simulink model "test_SimulinkMdl2_qLPVMPCbeta_UIO_testOL2"  (R2019b)
settings: Solver=FixedStepAuto  StartTime=0.0  StopTime=400  FixedStep=DT  RelTol=1e-3
values from neighbouring files (symbols this model uses):
  beta = [-0.13962634015954636; -0.1361356816555577; -0.13264502315156904;          -0.12915436464758037; -0.12566370614359171; -0.12217304763960307;          -0.11868238913561441; -0.11519173063162574; -0.11170107212763709;          -0.10821041362364842; -0.10471975511965977; -0.10122909661567112;          -0.097738438111682452; -0.094247779607693788; -0.09075712110370511;          -0.087266462599716474;  ...(+3598 chars)    [MdlMFile.m]
  betaLUT = 0.0 0.064193209888351435 0.11259119004615419 0.14929546421559495 0.18081611050661253 0.20926497731412011 0.23701571242082992 0.26197392072434883 0.28536133270107289 0.30770154712660031 0.32934362985133 0.35028758087526196 0.37035886727319672 0.38973202197033374 0.40858157789187255    [DD_test.sldd]    (also in exUIO_WECS.m = unique(Lin_points.Pitch))
  Cq = saveVarsMat.Cq    [MdlMFile.m]
  Ct = saveVarsMat.Ct    [MdlMFile.m]
  DT = 0.008    [LUTMFile.m]    (also in UIOLinestTr.m; exUIO_WECS.m; getFictInputMatricesOrd3M.m; initWorkspace.m)
  in1 = [Tr,Tg]    [UIOLinestTr.m]    (also in exUIO_WECS.m = [d,u1,u2])
  lambda = [0; 0.1; 0.2; 0.30000000000000004; 0.4; 0.5; 0.60000000000000009;            0.70000000000000007; 0.8; 0.9; 1; 1.1; 1.2000000000000002; 1.3;            1.4000000000000001; 1.5; 1.6; 1.7000000000000002; 1.8; 1.9000000000000001;            2; 2.1; 2.2; 2.3000000000000003; 2.4000000000000004; 2.5; 2.6;            2.7; 2.8000000000000003; 2.9000000000000004; 3; 3.1; 3.2; 3.3000000000000003;            ...(+1285 chars)    [MdlMFile.m]    (also in exLQR_hamiltonian.m = -10; koopmanKhalil.m = 1)
  lambdaCqVecLUT = 0.0 6.127061506348616E-5 0.00012254123012697232 0.00018381184519045848 0.00024508246025394464 0.00030635307531743077 0.00036762369038091696 0.00042889430544440315 0.00049016492050788928 0.00055143553557137541 0.00061270615063486154 0.00067397676569834778 0.00073524738076183392 0.00079651799582532 0.00085778861088880629 0.00091905922595229242 0.00098032984101577856 0.0010416004560792648 0.001102871    [DD_test.sldd]    (also in exUIO_WECS.m = lambdaCqVecMin : dLlambdaCqVec:lambdaCqVecMax)
  lambdaTildaMat = 14.419529569316524 14.349603210880673 12.133085869773012 9.9 8.4 7.3000000000000007 6.5 5.8000000000000007 5.4 4.9 4.6000000000000005 4.3 4.1000000000000005 3.9000000000000004 3.7 13.719392614649337 13.574357234178933 11.313379017594022 9.2598290519250313 7.9268106449449158 6.9824653636911407 6.2259000594299776 5.6530125740384722 5.1921371802911152 4.81807621242771 4.4910785109643978 4.22716815598    [DD_test.sldd]    (also in exUIO_WECS.m = lambdaCqVecMax *ones(size(lambdaCqMat)))
  Lin_points = 0.74811652133345019 0.78122947334555715 0.82586806925039735 0.88042797952230989 0.94564154658981237 1.06231329175348 1.1780905557148451 1.2402773842094346 1.254474305465946 1.2544764615597244 1.2544775037226534 1.2544778841663968 1.2544780221694662 1.2544779823335293 1.254477987181289 1.2544781738200332 1.254478189259095 1.2544780953600987 1.2544781548505395 1.2544783366942183 1.2544785605869417 1    [DD_test.sldd]    (also in LinPointsMFile.m = struct)
  multTau = 0.02    [UIOLinestTr.m]    (also in exUIO_WECS.m = 1)
  rho = 1.2250    (= 1.225)    [ABqL_WT_est_matlab.m]    (also in MdlMFile.m; UIOLinestTr.m; getFictInputMatricesOrd3M.m; testTorqueFromomegaNonLin.m)
  sysEst = c2d(ss(F,[T*B,K],eye(nx),[zeros(size(T*B)),H]),DT,'zoh')    [exUIO_WECS.m]
  wecs = 3.0    [DD_test.sldd]    (also in MdlMFile.m = struct)
  x0 = [0,Lin_points.RSpeed(idxNearestV1),Lin_points.RSpeed(idxNearestV1)]'    [UIOLinestTr.m]    (also in exUIO_WECS.m = x0([1:idxS,end]))
undefined symbols (not defined in the file or in its folder): Rotor_Lambda
libraries: sharedTrackingLibrary x1
(part 2 of 2)

== matlab function test_SimulinkMdl2_qLPVMPCbeta_UIO_testOL2/MATLAB Function ==
  settings: updateMethod=DISCRETE
  data: rhoP input; lambda input; beta input; Cq input; A output; Bout output; DT input; ytdot input; zetadot input
function [A,Bout] = ABqL_WT_beta_m(rhoP,lambda,beta,Cq,DT,ytdot,zetadot)
% ABqL calculates system (A) and input (B) matrix for quasiLPV
% representation for ve
%
% Inputs: * Ts: Sampling time
%         * AwithV: Scheduling parameter vector: AwithV = V
%
% Outputs: * A: System matrix A(AwithV) at current estimated air speed AwithV, discretised with Ts
%          * B: Input matrix B(AwithV) at current AwithV, discretised with Ts

% Pablo S.G. Cisneros, Herbert Werner, ICS TUHH
% modified for WECS simulation: Antje Dittmer

persistent lambdaVec pitchVec CqVec Cqdlambda Cqdbeta

if isempty(lambdaVec)
    lambdaVec =  lambda;
    pitchVec = beta;
    CqVec = Cq;
    %% Compute gradients %%[Cpdlambda,Cpdbeta] = gradient(Cp,mean(diff(Xq(1,:))),mean(diff(Yq(:,1))));
    [Cqdlambda,Cqdbeta] = gradient(CqVec,mean(diff(lambda)),mean(diff(beta))); %dcQ/dbetaDeg * dbetaDeg/dbetaRad *betaRAd
end

rb = 63;
%% Parameters
if length(rhoP) == 1
    
    Vbar = rhoP - zetadot*rb - ytdot;
    LUT_V = 4:25; % LUT table rows
    
    LUT_omega = ...%[0.4815, 0.6017,0.7217,0.8413,0.9603,1.0786,1.1949, repmat(1.2671,1,15)];
        [0.7458832277625318 0.77759738173519954 0.820732502042672 ...
        0.87379091011167287 0.93538972625666472 1.0429417531956238 ...
        1.1591854391157337 1.2371015764176956 1.2554479267196832 ...
        1.2547857982936621 1.2545286368009017 1.2546177195393646 ...
        1.2545376249695805 1.2545426663335242 1.2545426663335242 ...
        1.2545426663335242 1.2545426663335242 1.2545426663335242 ...
        1.2545426663335242 1.2545426663335242 1.2545426663335242 ...
        1.2545426663335242];
    
    LUT_beta =  [0 0 0 0 0 0 0 0 0.064193209888351435 0.11259119004615419 ...
        0.14929546421559495 0.18081611050661253 0.20926497731412011 ...
        0.23701571242082992 0.26197392072434883 0.28536133270107289 ...
        0.30770154712660031 0.32934362985133 0.35028758087526196 ...
        0.37035886727319672 0.38973202197033374 0.40858157789187255 ...
        ];
    
    
    % Get omegabar and beta
    omegabar = interp1(LUT_V,LUT_omega,Vbar,'pchip');
    beta_bar = interp1(LUT_V,LUT_beta,Vbar,'pchip');
    
elseif length(rhoP) == 3
    % rho = xdotk_1([1,3,4]); % Tg not included: [Omega [1/s], beta[rad], V [m/s]];
    Vbar = rhoP(3)- zetadot*rb - ytdot;
    omegabar = rhoP(1); % pass OmegaR OmegaG/Ng as approximation of omegaR
    beta_bar = rhoP(2);
    
else
    error('Unexpected length of scheduling parameter rho')
end

%% Physical and model constants
rho = 1.2250;
rb = 63; % m blade radius
Ng = 97; %Gearbox ratio
Jr = (115926 + 3 * 11.776e6) *1; %kg*m^2 Inertia of the rotor (Hub inertia + 3 blades
Jg = 534.116;% * Ng^2; %kg*m^2 Inertia of the generator (HSS)
Jgr = Jg * Ng^2; % Inertia of the generator in LSS
Ks = 867637000; %Nm/rad Stiffness of the transmission
Bs = 6215000;  %Nm/rad/sec        %Damping of the transmission
tau_g = 0.01; % for pitch actuator and airspeed

%% Lambda
Lambda_bar = omegabar*rb/Vbar;
dlambdadomega= rb/Vbar;
dlambdadV = - omegabar*rb/Vbar^2;

%% Grid points
Cqb = interp2(lambdaVec,pitchVec,Cq,Lambda_bar,beta_bar);
dCqdlambdab = interp2(lambdaVec,pitchVec,Cqdlambda,Lambda_bar,beta_bar);
dCqdbetab = interp2(lambdaVec,pitchVec,Cqdbeta,Lambda_bar,beta_bar);
%% Tr=0.5*pi*rb^3*Cq*v^2
dTrdomega = 0.5*rho*pi*rb^3*(dCqdlambdab*dlambdadomega)*Vbar^2;% br = dTr/domega
dTrdbeta = 0.5*rho*pi*rb^3*dCqdbetab*Vbar^2;% Krb = dTr/dbeta
dTrdV =  2*0.5*rho*pi*rb^3*Vbar*Cqb + ...
    0.5*rho*pi*rb^3*Vbar^2*dCqdlambdab*dlambdadV;

%% Create system matrix A:
% States: [Theta_s [rad], omega_r [rad/s], omega_gr [rad/s], T_g [Nm]]
% States for model xA = [y, xdot] with y = [Tg, beta]
% x = [ThetaS, OmegaR, OmegaG, Tg, beta,]
Atemp = [[0,1,-1,0] ;
    [-Ks/Jr, (-Bs + dTrdomega)/Jr, Bs/Jr,0];
    Ks/Jgr, Bs/Jgr, -Bs/Jgr, -Ng/Jgr;
    zeros(1,3), -1/tau_g];

%% Create input matrix B
% Input orig model: V [m/s], T_g_ref [Nm], beta [rad],
% -> vel model: Vdot [m/s^2]  , T_g_refDot [Nm/s]
% for beta: Vdot [m/s^2]  T_g_refDot [Nm/s] betaDot [rad/s],
Btemp = [zeros(1,3); dTrdV/Jr, 0 dTrdbeta/Jr; zeros(1,3);  0,  1/tau_g,0];

% With Beta
Aeval = [Atemp,Btemp(:,3); zeros(1, size(Atemp,2)), -1/tau_g];
Beval = [Btemp; zeros(1, size(Btemp,2))];
Beval(:,3) = 0;
Beval(end,3) = 1/tau_g;


%% Check rank
Bu = Beval(:,2:3);
Bd = Beval(:,1);
nxEval = size(Aeval,2);

% Also create an additional state for the disturbance
tau1 =  1/DT *0.1;
A =[[Aeval, zeros(nxEval,1)]; [zeros(1,nxEval),-tau1]];
E = [Bd;tau1]; %xd_dot = -xd + Ed
B = [Bu; zeros(1,2)];
Bout = [E,B];
%fprintf('rank(C*E) is %d; rank(E) is %d\n', rank(C1*E1),rank(E1));


%% Calculate observer matrices
% Ceval = [zeros(nxEval-1,1),eye(nxEval-1)]; %
% nyEval = size(Ceval,1);

%C = [Ceval, zeros(nyEval,1)]; %[zeros(1,nx),1]];
% H = E*inv((C*E)'*(C*E))*(C*E)'; %#ok<MINV,*NOPTS> display output, inv is fast enough
% nx = size(A,1);
% T = eye(nx)-H*C;
% A1 = T*A;

% Pole placement with Q and R
% Qe = eye(nxEval); %B*B'; %
% Re = C*C';
% K1 = lqr(A',C',Qe,Re)';
%
% % Calculate F and K
% F = A1 - K1*C; %T*A -K1*C
% K = K1 + F*H;
% T = eye(size(H*C)) - H*C;

% Sys with no ctrl input: xdot = Ax + Ed, y = Cx
% nd = size(E,2); %nu = 0;
%sys = ss(A,[E,B],C,zeros(ny,nd+2));

end

== matlab function test_SimulinkMdl2_qLPVMPCbeta_UIO_testOL2/MATLAB Function2 ==
  settings: updateMethod=DISCRETE
  data: B1 output; A1 output; uLin output; wind input; Tg input; pitch input; lambda input; beta input; Cq input; Ct input; DT input; omegabar input; ytdot input; zetadot input
function [B1,A1,uLin] = getFictInputMatrices(wind,Tg,pitch,lambda,beta,Cq,Ct,DT,omegabar,ytdot,zetadot)
% getTrFt
% representation for ve
%
% Inputs: * Ts: Sampling time
%         * AwithV: Scheduling parameter vector: AwithV = V
%
% Outputs: * A: System matrix A(AwithV) at current estimated air speed AwithV, discretised with Ts
%          * B: Input matrix B(AwithV) at current AwithV, discretised with Ts

% Pablo S.G. Cisneros, Herbert Werner, ICS TUHH
% modified for WECS simulation: Antje Dittmer

persistent lambdaVec pitchVec CqVec CtVec% Cqdlambda Cqdbeta

if isempty(lambdaVec)
    lambdaVec =  lambda;
    pitchVec = beta;
    CqVec = Cq;
    CtVec = Ct;
    %% Compute gradients %%[Cpdlambda,Cpdbeta] = gradient(Cp,mean(diff(Xq(1,:))),mean(diff(Yq(:,1))));
    %[Cqdlambda,Cqdbeta] = gradient(CqVec,mean(diff(lambda)),mean(diff(beta))); %dcQ/dbetaDeg * dbetaDeg/dbetaRad *betaRAd
end

%% Physical and turbine model constants
rho = 1.2250; % air density
N = 3;% Number of blades
Ng = 97; % Gearbox ratio
mh = 56780; % kg;  Hub mass
mb = 0.25*17740; %kg;  Modal mass of each blade
mn = 240000; % kg;  Nacellle mass
mtower = 347460;% kg; Mass of the tower and nacelle
mt = 0.25*mtower + mn + mh;
H =  87.6;

Jg = 534.116; %  kg*m^2; Inertia of the generator
Jr = 115926 + 3 * 11.776e6; % kg*m^2; Inertia of the rotor (Hub inertia + 3 blades)
f0 = 0.324; % Hz, First natural tower fore-aft frequency
% f0sw = 0.3120; % First natural tower sidewards frequency
wnb = 0.6993 * 2*pi; % rad/s First natural blade frequency 
wnt = f0 * 2*pi; % wnb; 0.3240
zetat = 1/100; %damping ratio of tower (Table 6.2)
zetab = 0.477465/100;% damping ratio of blade

Kt = wnt^2 * mt; % Stiffness of the tower s^2 + B/Ms + K/m
Bt = 2 * zetat * wnt *mt; % tower 2*6421;

Kb = wnb^2 * mb; %Stiffness of each blade
Bb = 2 * zetab* wnb *mb; %Damping of the blade
Ks = 867637000; %Nm/rad Stiffness of the transmission % 2*zeta*wn = B
Bs = 6215000;  %Nm/rad/sec %Damping of the transmission
rb = 63; % m blade radius
% etag = 0.944; %Drivetrain.Generator.Efficiency: 0.944;

%% Effective wind speed and lambda
Vbar = wind - zetadot*rb - ytdot;
Lambda_bar = omegabar*rb/Vbar;

%% Grid points
Cqb = interp2(lambdaVec,pitchVec,CqVec,Lambda_bar,pitch);
Ctb = interp2(lambdaVec,pitchVec,CtVec,Lambda_bar,pitch);

%% 
Tr = 0.5*rho*pi*rb^3*Cqb*Vbar^2;% br = dTr/domega
Ft = 0.5*rho*pi*rb^2*Ctb*Vbar^2;% br = dTr/domega
uLin = [Ft,Tr*(3/(2*H)),Tr,Tg]';

%% Lagrange's Model matrices
% Force input w = [Ft_fa,Ft_sw,Tr,Tg]; Ft_fa = Ft, Ft_sw = 3/2*Tg
% States q: xdot_fa, zeta, xdot_sw, omega_r, omega_gr
M =[mt+N*mb N*mb*rb 0 0 0; % 
    N*mb*rb  N*mb*rb^2 0 0 0;
    0 0 mt 0 0;
    0 0 0 Jr 0;
    0 0 0 0 Jg*Ng^2];

Ce = [Bt 0 0 0 0;
    0 N*Bb*rb^2 0 0 0 ; %
    0 0 Bt 0 0
    0 0 0  Bs -Bs;
    0 0 0 -Bs Bs];

K = [Kt 0 0 0;
    0 N*Kb*rb^2 0 0; %
    0 0 Kt 0
    0 0 0 Ks;
    0 0 0 -Ks];

Q = [1 0 0 0;
    rb 0 0 0;
    0 1 0 0;
    0 0 1 0;
    0 0 0 -Ng];

L = [eye(4), [0;0;0;-1]];

A1 = [zeros(4), L;...
    -M\K, -M\Ce];
B1 = [zeros(4); M\Q];

%% Discretize Matrices
%% Calculate discrete forms of A,B
% A2 = A1*A1;
% A3 = A1*A2;
% Apre = (1.0/24.0)*DT^4*A3+(1.0/6.0)*DT^3*A2+0.5*DT^2*Arho+DT*eye(size(Arho));
% 
% %% Finish calculation of A,B
% Ak = Apre*A1 + eye(size(A1));
% Bk = Apre*B1;




% 
% x0 = [0,0,0,






% 
% 
% dCqdlambdab = interp2(lambdaVec,pitchVec,Cqdlambda,Lambda_bar,beta_bar);
% dCqdbetab = interp2(lambdaVec,pitchVec,Cqdbeta,Lambda_bar,beta_bar);
% %% Tr=0.5*pi*rb^3*Cq*v^2
% dTrdomega = 0.5*rho*pi*rb^3*(dCqdlambdab*dlambdadomega)*Vbar^2;% br = dTr/domega
% dTrdbeta = 0.5*rho*pi*rb^3*dCqdbetab*Vbar^2;% Krb = dTr/dbeta
% dTrdV =  2*0.5*rho*pi*rb^3*Vbar*Cqb + ...
%     0.5*rho*pi*rb^3*Vbar^2*dCqdlambdab*dlambdadV;
% 
% %% Create system matrix A:
% % States: [Theta_s [rad], omega_r [rad/s], omega_gr [rad/s], T_g [Nm]]
% % States for model xA = [y, xdot] with y = [Tg, beta]
% % x = [ThetaS, OmegaR, OmegaG, Tg, beta,]
% Atemp = [[0,1,-1,0] ;
%     [-Ks/Jr, (-Bs + dTrdomega)/Jr, Bs/Jr,0];
%     Ks/Jgr, Bs/Jgr, -Bs/Jgr, -Ng/Jgr;
%     zeros(1,3), -1/tau_g];
% 
% %% Create input matrix B
% % Input orig model: V [m/s], T_g_ref [Nm], beta [rad],
% % -> vel model: Vdot [m/s^2]  , T_g_refDot [Nm/s]
% % for beta: Vdot [m/s^2]  T_g_refDot [Nm/s] betaDot [rad/s],
% Btemp = [zeros(1,3); dTrdV/Jr, 0 dTrdbeta/Jr; zeros(1,3);  0,  1/tau_g,0];
% 
% % With Beta
% Aeval = [Atemp,Btemp(:,3); zeros(1, size(Atemp,2)), -1/tau_g];
% Beval = [Btemp; zeros(1, size(Btemp,2))];
% Beval(:,3) = 0;
% Beval(end,3) = 1/tau_g;
% 
% 
% %% Check rank
% Bu = Beval(:,2:3);
% Bd = Beval(:,1);
% nxEval = size(Aeval,2);
% 
% % Also create an additional state for the disturbance
% tau1 =  1/DT *0.1;
% A =[[Aeval, zeros(nxEval,1)]; [zeros(1,nxEval),-tau1]];
% E = [Bd;tau1]; %xd_dot = -xd + Ed
% B = [Bu; zeros(1,2)];
% Bout = [E,B];
% 
% end
% 
% % %% Parameters
% % if length(rhoP) == 1
% %     Vbar = rhoP; % Vbar
% %     LUT_V = 4:25; % LUT table rows
% %
% %     LUT_omega = ...%[0.4815, 0.6017,0.7217,0.8413,0.9603,1.0786,1.1949, repmat(1.2671,1,15)];
% %         [0.7458832277625318 0.77759738173519954 0.820732502042672 ...
% %         0.87379091011167287 0.93538972625666472 1.0429417531956238 ...
% %         1.1591854391157337 1.2371015764176956 1.2554479267196832 ...
% %         1.2547857982936621 1.2545286368009017 1.2546177195393646 ...
% %         1.2545376249695805 1.2545426663335242 1.2545426663335242 ...
% %         1.2545426663335242 1.2545426663335242 1.2545426663335242 ...
% %         1.2545426663335242 1.2545426663335242 1.2545426663335242 ...
% %         1.2545426663335242];
% %
% %     LUT_beta =  [0 0 0 0 0 0 0 0 0.064193209888351435 0.11259119004615419 ...
% %         0.14929546421559495 0.18081611050661253 0.20926497731412011 ...
% %         0.23701571242082992 0.26197392072434883 0.28536133270107289 ...
% %         0.30770154712660031 0.32934362985133 0.35028758087526196 ...
% %         0.37035886727319672 0.38973202197033374 0.40858157789187255 ...
% %         ];
% %
% %
% %     % Get omegabar and beta
% %     omegabar = interp1(LUT_V,LUT_omega,Vbar,'pchip');
% %     beta_bar = interp1(LUT_V,LUT_beta,Vbar,'pchip');
% %
% % elseif length(rhoP) == 3
% %     % rho = xdotk_1([1,3,4]); % Tg not included: [Omega [1/s], beta[rad], V [m/s]];
% %     Vbar = rhoP(3);
% %     omegabar = rhoP(1); % pass OmegaR OmegaG/Ng as approximation of omegaR
% %     beta_bar = rhoP(2);
% %
% % else
% %     error('Unexpected length of scheduling parameter rho')
% % end

== matlab function test_SimulinkMdl2_qLPVMPCbeta_UIO_testOL2/MATLAB Function1 ==
  data: Tr input; omegaR input; lambdaFunTr output
function lambdaFunTr = getlambdaFunTr(Tr,omegaR)

rho = 1.2250; % air density
rb = 63; % m blade radius

lambdaFunTr = 2* Tr /(rho *pi * rb^5*omegaR^2);


% %% Constants

% 
% %% Calculations
% CqPitch = interp2(lambda,beta,Cq,lambda,pitch);
% lambdaCqFun = (lambda .^ (-2)) .* CqPitch';
% 
% 
% %% To estimate the aerodynamic Torque Tr, use the equation
% %      Tr = 0.5 *rho *pi*R^3 *C_Q *V^2
% %         = 0.5 *rho *pi*R^3 *C_Q *(omegaR^2*R^2/lambda^2)
% % =>  2* Tr /(rho *pi * R^5 omegaR^2) = lambda^(-2) C_Q
% 
% lambdaFunTr = 2* Tr /(rho *pi * rb^5*omegaR^2);
% % diffLambda = abs(lambdaCqFun - lambdaFunTr); % difference to LUT pitch vector
% % idxNearestLambda =  min(diffLambda) == diffLambda; % index of nearest pitch
% 
% lambdaTilda = interp1(lambdaCqFun,lambda,lambdaFunTr);
% vTilda = omegaR * rb/lambdaTilda;

== matlab function test_SimulinkMdl2_qLPVMPCbeta_UIO_testOL2/Subsystem2/MATLAB Function3 ==
  data: omegaR input; Tr input; lambdaFunTr output
function lambdaFunTr = getLambdaFunTr(omegaR,Tr)
% calculate the lambda^(-2) Cq(beta,lambda) at rotor speed and torque 

%% Parameters
rho = 1.2250; % air density
rb = 63; % m blade radius

%% Calculation
lambdaFunTr = 2* Tr /(rho *pi * rb^5*omegaR^2);

== matlab function test_SimulinkMdl2_qLPVMPCbeta_UIO_testOL2/MATLAB Function3 ==
  settings: updateMethod=DISCRETE
  data: B1 output; A1 output; uLin output; wind input; Tg input; pitch input; lambda input; beta input; Cq input; Ct input; DT input; omegabar input; ytdot input; zetadot input; Bout output; Aout output
function [B1,A1,uLin, Bout, Aout] = getFictInputMatricesOrd3(wind,Tg,pitch,lambda,beta,Cq,Ct,DT,omegabar,ytdot,zetadot)
% getTrFt
% representation for ve
%
% Inputs: * Ts: Sampling time
%         * AwithV: Scheduling parameter vector: AwithV = V
%
% Outputs: * A: System matrix A(AwithV) at current estimated air speed AwithV, discretised with Ts
%          * B: Input matrix B(AwithV) at current AwithV, discretised with Ts

% Pablo S.G. Cisneros, Herbert Werner, ICS TUHH
% modified for WECS simulation: Antje Dittmer

persistent lambdaVec pitchVec CqVec CtVec Cqdlambda Cqdbeta

if isempty(lambdaVec)
    lambdaVec =  lambda;
    pitchVec = beta;
    CqVec = Cq;
    CtVec = Ct;
    %% Compute gradients %%[Cpdlambda,Cpdbeta] = gradient(Cp,mean(diff(Xq(1,:))),mean(diff(Yq(:,1))));
    [Cqdlambda,Cqdbeta] = gradient(CqVec,mean(diff(lambda)),mean(diff(beta))); %dcQ/dbetaDeg * dbetaDeg/dbetaRad *betaRAd
end

%% Physical and turbine model constants
rho = 1.2250; % air density
N = 3;% Number of blades
Ng = 97; % Gearbox ratio
mh = 56780; % kg;  Hub mass
mb = 0.25*17740; %kg;  Modal mass of each blade
mn = 240000; % kg;  Nacellle mass
mtower = 347460;% kg; Mass of the tower and nacelle
mt = 0.25*mtower + mn + mh;
H =  87.6;

Jg = 534.116; %  kg*m^2; Inertia of the generator
Jr = 115926 + 3 * 11.776e6; % kg*m^2; Inertia of the rotor (Hub inertia + 3 blades)
Jgr = Jg * Ng^2; % Inertia of the generator in LSS
f0 = 0.324; % Hz, First natural tower fore-aft frequency
% f0sw = 0.3120; % First natural tower sidewards frequency
wnb = 0.6993 * 2*pi; % rad/s First natural blade frequency 
wnt = f0 * 2*pi; % wnb; 0.3240
zetat = 1/100; %damping ratio of tower (Table 6.2)
zetab = 0.477465/100;% damping ratio of blade

Kt = wnt^2 * mt; % Stiffness of the tower s^2 + B/Ms + K/m
Bt = 2 * zetat * wnt *mt; % tower 2*6421;

Kb = wnb^2 * mb; %Stiffness of each blade
Bb = 2 * zetab* wnb *mb; %Damping of the blade
Ks = 867637000; %Nm/rad Stiffness of the transmission % 2*zeta*wn = B
Bs = 6215000;  %Nm/rad/sec %Damping of the transmission
rb = 63; % m blade radius
% etag = 0.944; %Drivetrain.Generator.Efficiency: 0.944;

%% Effective wind speed and lambda
Vbar = wind - zetadot*rb - ytdot;
Lambda_bar = omegabar*rb/Vbar;
dlambdadomega = rb/Vbar;
dlambdadV = - omegabar*rb/Vbar^2;
beta_bar = pitch;

%% Grid points
Cqb = interp2(lambdaVec,pitchVec,CqVec,Lambda_bar,beta_bar);
dCqdlambdab = interp2(lambdaVec,pitchVec,Cqdlambda,Lambda_bar,beta_bar);
dCqdbetab = interp2(lambdaVec,pitchVec,Cqdbeta,Lambda_bar,beta_bar);
Tr = 0.5*rho*pi*rb^3*Cqb*Vbar^2;% br = dTr/domega
%Ft = 0.5*rho*pi*rb^2*Ctb*Vbar^2;% br = dTr/domega

%% Tr=0.5*pi*rb^3*Cq*v^2
dTrdomega = 0.5*rho*pi*rb^3*(dCqdlambdab*dlambdadomega)*Vbar^2;% br = dTr/domega
dTrdbeta = 0.5*rho*pi*rb^3*dCqdbetab*Vbar^2;% Krb = dTr/dbeta
dTrdV =  2*0.5*rho*pi*rb^3*Vbar*Cqb + ...
    0.5*rho*pi*rb^3*Vbar^2*dCqdlambdab*dlambdadV;

%% Lagrange's Model matrices
% Force input w = [Ft_fa,Ft_sw,Tr,Tg]; Ft_fa = Ft, Ft_sw = 3/2*Tg
% States q: xdot_fa, zeta, xdot_sw, omega_r, omega_gr
vecOmega = 4:5; 
Mall =[mt+N*mb N*mb*rb 0 0 0; % 
    N*mb*rb  N*mb*rb^2 0 0 0;
    0 0 mt 0 0;
    0 0 0 Jr 0;
    0 0 0 0 Jg*Ng^2];
M = Mall(vecOmega,vecOmega);

Ceall = [Bt 0 0 0 0;
    0 N*Bb*rb^2 0 0 0 ; %
    0 0 Bt 0 0
    0 0 0  Bs -Bs;
    0 0 0 -Bs Bs];
Ce = Ceall(vecOmega,vecOmega);

Kall = [Kt 0 0 0;
    0 N*Kb*rb^2 0 0; %
    0 0 Kt 0
    0 0 0 Ks;
    0 0 0 -Ks];
K = Kall(vecOmega,vecOmega(1));


Qall = [1 0 0 0;
    rb 0 0 0;
    0 1 0 0;
    0 0 1 0;
    0 0 0 -Ng];
Q = Qall(vecOmega,vecOmega-1);

Lall = [eye(4), [0;0;0;-1]];
L = Lall(vecOmega(1),vecOmega);
%L(vecOmega,vecOmega(1)) = Lall;

nqt = size(L,1);
A1 = [zeros(nqt), L;...
    -M\K, -M\Ce];
B1 = [zeros(size(L)); M\Q];


uLin = [Tr,Tg]';

%% Create system matrix A:
% States: [Theta_s [rad], omega_r [rad/s], omega_gr [rad/s], T_g [Nm]]
% States for model xA = [y, xdot] with y = [Tg, beta]
% x = [ThetaS, OmegaR, OmegaG, Tg, beta,]
Atemp = [[0,1,-1];
    [-Ks/Jr, (-Bs + dTrdomega)/Jr, Bs/Jr,];
    Ks/Jgr, Bs/Jgr, -Bs/Jgr];

%% Create input matrix B
% Input orig model: V [m/s], T_g_ref [Nm], beta [rad],
% -> vel model: Vdot [m/s^2]  , T_g_refDot [Nm/s]
% for beta: Vdot [m/s^2]  T_g_refDot [Nm/s] betaDot [rad/s],
Btemp = [zeros(1,3); dTrdV/Jr, 0 dTrdbeta/Jr;  0,  -Ng/Jgr,0];

%% Check rank
Bu = Btemp(:,2:3);
Bd = Btemp(:,1);
nxEval = size(Atemp,2);

% Also create an additional state for the disturbance
tau1 =  1/DT;
Aout = [[Atemp, zeros(nxEval,1)]; [zeros(1,nxEval),-tau1]];
E = [Bd;tau1]; %xd_dot = -xd + Ed
B = [Bu; zeros(1,2)];
Bout = [E,B];

%% Discretize Matrices
%% Calculate discrete forms of A,B
% A2 = A1*A1;
% A3 = A1*A2;
% Apre = (1.0/24.0)*DT^4*A3+(1.0/6.0)*DT^3*A2+0.5*DT^2*Arho+DT*eye(size(Arho));
% 
% %% Finish calculation of A,B
% Ak = Apre*A1 + eye(size(A1));
% Bk = Apre*B1;
